simulink model "DesignModel"  (R2025a)
settings: Solver=VariableStepAuto  StartTime=0.0  StopTime=10.0  RelTol=1e-3
values from neighbouring files (symbols this model uses):
  K_1 = L_1 / J_p    (= 0.518122400475)    [init_heli_3_10.m]    (also in init_heli_part3.m)
  K_pd = -(lambda_1 + lambda_2) / K_1    (= 7.72018348624)    [init_heli_part3.m]    (also in simDesignModel.m = -(lambda_1 + lambda_2) / K_1)
  K_pp = (lambda_1 * lambda_2) / K_1    (= 7.72018348624)    [init_heli_part3.m]    (also in simDesignModel.m = (lambda_1 * lambda_2) / K_1)
settings Model: Creator=ole  LastModifiedBy=ole

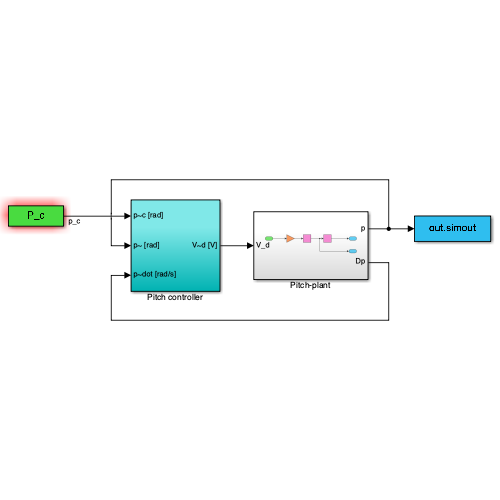
[thumbnail: Simulink's stored preview of the top-level diagram]
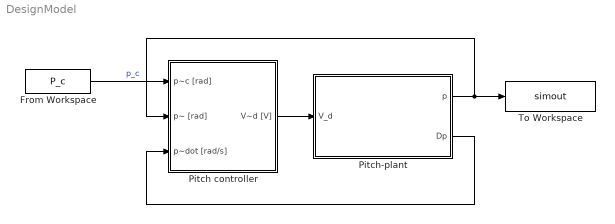
== system DesignModel ==
  From Workspace : FromWorkspace  VariableName=P_c
  Pitch controller : Subsystem
  Pitch-plant : Subsystem
  To Workspace : ToWorkspace  VariableName=simout  SaveFormat=Timeseries  SampleTime=-1
  wires:
  Pitch controller/1(V~d [V]) -> Pitch-plant/1(V_d)
  Pitch-plant/1(p) -> Pitch controller/2(p~ [rad]), To Workspace/1
  Pitch-plant/2(Dp) -> Pitch controller/3(p~dot [rad/s])
  From Workspace/1 -> Pitch controller/1(p~c [rad])  "p_c"

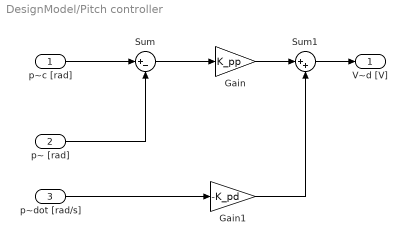
== system DesignModel/Pitch controller ==
  p~c [rad] : Inport
  p~ [rad] : Inport  Port=2
  p~dot [rad/s] : Inport  Port=3
  Gain : Gain  Gain=K_pp
  Gain1 : Gain  Gain=-K_pd
  Sum : Sum  Inputs=|+-
  Sum1 : Sum  Inputs=|++
  V~d [V] : Outport  InitialOutput=0
  wires:
  Sum/1 -> Gain/1
  p~ [rad]/1 -> Sum/2
  p~dot [rad/s]/1 -> Gain1/1
  Gain/1 -> Sum1/1
  Gain1/1 -> Sum1/2
  p~c [rad]/1 -> Sum/1
  Sum1/1 -> V~d [V]/1

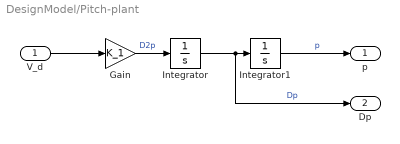
== system DesignModel/Pitch-plant ==
  V_d : Inport
  Gain : Gain  Gain=K_1
  Integrator : Integrator
  Integrator1 : Integrator
  p : Outport
  Dp : Outport  Port=2
  wires:
  Integrator1/1 -> p/1  "p"
  V_d/1 -> Gain/1
  Integrator/1 -> Dp/1, Integrator1/1  "Dp"
  Gain/1 -> Integrator/1  "D2p"
